simulink model "Quadcopter_Model"  (R2025b)
settings: Solver=ode8  StartTime=0.0  StopTime=10  FixedStep=0.01  RelTol=1e-3
InitFcn:
  | g = 9.81;
  | m = 2.4;
settings Model: Creator=MehrSystem  LastModifiedBy=MehrSystem
settings DebuggingCC: UnconnectedInputMsg=warning  UnconnectedOutputMsg=warning  UnconnectedLineMsg=warning
settings ModelReferenceCC: EnableRefExpFcnMdlSchedulingChecks=on
settings RTWCC: GPUComputeCapability=3.5  DLArmComputeVersion=19.05

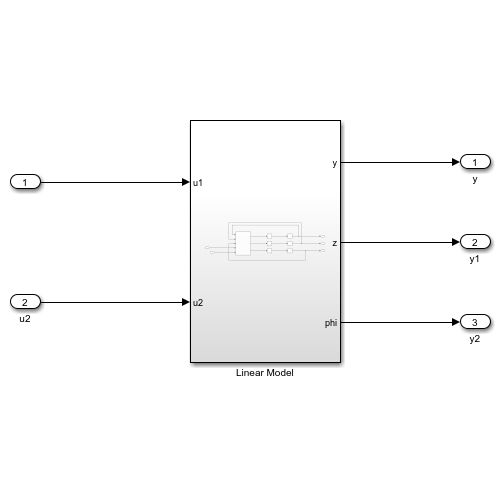
[thumbnail: Simulink's stored preview of the top-level diagram]
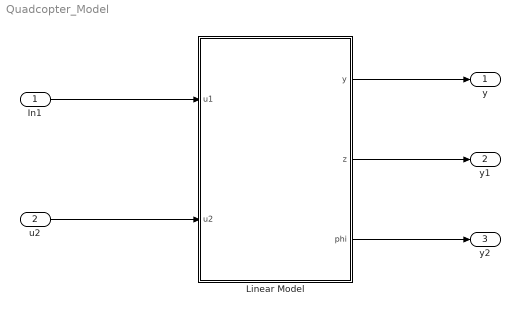
== system Quadcopter_Model ==
  In1 : Inport
  u2 : Inport  Port=2
  Linear Model : Subsystem
  y : Outport
  y1 : Outport  Port=2
  y2 : Outport  Port=3
  wires:
  In1/1 -> Linear Model/1(u1)
  u2/1 -> Linear Model/2(u2)
  Linear Model/1(y) -> y/1
  Linear Model/2(z) -> y1/1
  Linear Model/3(phi) -> y2/1

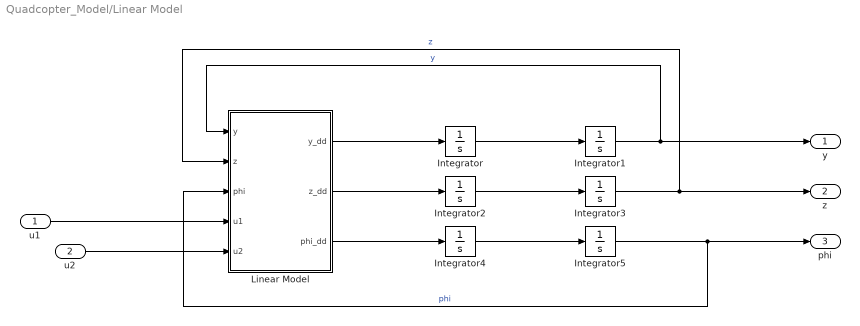
== system Quadcopter_Model/Linear Model ==
  u1 : Inport
  u2 : Inport  Port=2
  Integrator{,1..5} (6 alike) : Integrator
  Linear Model : MATLAB Function  TreatAsAtomicUnit=on
  y : Outport
  z : Outport  Port=2
  phi : Outport  Port=3
  wires:
  Integrator/1 -> Integrator1/1
  Integrator2/1 -> Integrator3/1
  Integrator3/1 -> z/1, Linear Model/2(z)  "z"
  Integrator1/1 -> y/1, Linear Model/1(y)  "y"
  Linear Model/1(y_dd) -> Integrator/1
  Integrator5/1 -> phi/1, Linear Model/3(phi)  "phi"
  Linear Model/2(z_dd) -> Integrator2/1
  u1/1 -> Linear Model/4(u1)
  u2/1 -> Linear Model/5(u2)
  Linear Model/3(phi_dd) -> Integrator4/1
  Integrator4/1 -> Integrator5/1

== matlab function Quadcopter_Model/Linear Model/Linear Model ==
  data: y input; z input; phi input; y_dd output; u1 input; z_dd output; phi_dd output; u2 input
function [y_dd,z_dd,phi_dd] = fcn(y, z, phi, u1, u2)
g = 9.81;
m = 2.4;
Ix = 0.04;
y_dd = -g*phi;
z_dd = -g + u1/m;
phi_dd = u2/Ix;
